simulink model "afe_inv_ttype_psm"  (R2026a)
settings: Solver=ode23tb  StopTime=simlength  FixedStep=tc  MaxStep=glb_time.tc
values from neighbouring files (symbols this model uses):
  afe_ctrl = ctrl_afe_setup(glb_time.ts_afe, grid_emu.omega_grid_nom)    [init_model.m]
  afe_pwm_phase_shift_mod1 = 0    [init_model.m]
  DThs_init = 0    [init_model.m]
  filters = setup_global_filters(glb_time.ts_afe, glb_time.ts_inv, glb_time.ts_dab, glb_time.tc)    [init_model.m]
  frt_data = frt_settings(test_index, test_subindex, asymmetric_error_type,      enable_frt_1, enable_frt_2, start_time_LVRT, deepPOSxi, deepPOSeta, deepNEGxi, deepNEGeta)    [init_model.m]
  glb_time = timing_setup(fpwm_afe, trgo_afe, fpwm_inv, trgo_inv, fpwm_single_phase_inv, trgo_single_phase_inv, fpwm_dab, trgo_dab,      fpwm_psfbc, trgo_psfbc, fpwm_isop_rail, trgo_isop_rail, fpwm_cllc, trgo_cllc, t_measure, tc_factor, tc_decimation, delay_pwm, dead_time_afe,      dead_time_inv, dead_time_single_phase_inv, dead_time_dab, dead_time_psfbc, dead_time_isop_rail, dead_time_cllc)    [init_model.m]
  grid_emu = grid_three_phase_emulator('Dyn11', delta_star, grid_nominal_power, application_voltage, us1, us2, fgrid,                  eq_grid_inductance, eq_grid_resistance, eta, ucc, i1m, p_iron, n1, n2, core_area, core_length, mur,                  up_xi_pu_ref, up_eta_pu_ref, un_xi_pu_ref, un_eta_pu_ref)    [init_model.m]
  i_react_pos_ref_2 = -ixi_ref_mod1*tan(acos(0.95))    [init_model.m]
  i_react_pos_ref_3 = ixi_ref_mod1*tan(acos(0.95))    [init_model.m]
  ixi_ref_mod1 = -0.85    [init_model.m]
  ki_align = 18    [init_model.m]
  kp_align = 0.25    [init_model.m]
  lim_down_align = -0.05    [init_model.m]
  lim_up_align = 0.05    [init_model.m]
  mavarage_filter_frequency_base_order = 2    [init_model.m]
  omega_m_sim = psm.omega_m_bez    [init_model.m]
  psm = psm_calculus()    [init_model.m]
  psm_ctrl = ctrl_pmsm_setup(glb_time.ts_inv, psm.omega_bez, u_psm_scale, psm.Jm_norm)    [init_model.m]
  simlength = 1.75    [init_model.m]
  Tambient = 40    [init_model.m]
  time_aux_power_supply_fault = 1e3    (= 1000)    [init_model.m]
  time_gain_afe_module_1 = 1.0002    [init_model.m]
  time_gain_inv_module_2 = 1.001    [init_model.m]
  time_i_react_pos_ref_1 = start_time_LVRT + error_length + 0.335    [init_model.m]
  time_i_react_pos_ref_2 = time_i_react_pos_ref_1 + 0.5    (= 0.5)    [init_model.m]
  time_start_motor_control = 0.25    [init_model.m]
  torque_overload_factor = 1    [init_model.m]
  u_cm_comp_mod1 = 0    [init_model.m]
  u_psm_scale_ekf = sqrt(3)/2 * 2/3 * hwdata.inv.udc_nom/psm.ubez    [init_model.m]
undefined symbols (not defined in the file or in its folder): hwdata, magnitude, omega_m_bez, rpm_base, torque_base
libraries: fl_lib x74, nesl_utility x43, moving_average_filter x10, moving_average_filter_cc x8, discrete_time_low_pass_filter x4, sl_discontinuities x3, single_phase_transformer_lib x3, linear_double_integrator_observer_ccaller x2, threephase_inductor_lib x2, dclink_for_three_levels x2, three_phase_three_level_ttype_inverter_ideal_switch_based_model x2, cstblocks_lti x2
(part 9 of 9)

== matlab function afe_inv_ttype_psm/afe_abc_inv_psm_mod1/inv_psm_mod1/inverter/deadtime_generator_for_ttype/dead_time_generator_cmos_simulink_phv/dead_time_leg_generator_1/MATLAB Function3 ==
  data: u input; y output; Vpos_rail_dtg parameter
function y = not_cmos(u, Vpos_rail_dtg)

vth = Vpos_rail_dtg/2;

if u > vth
    y = 0;
else
    y = Vpos_rail_dtg;
end

== matlab function afe_inv_ttype_psm/afe_abc_inv_psm_mod1/inv_psm_mod1/inverter/deadtime_generator_for_ttype/dead_time_generator_cmos_simulink_phv/dead_time_leg_generator_1/MATLAB Function4 ==
  data: u1 input; u2 input; y output; Vpos_rail_dtg parameter
function y = and_cmos(u1, u2, Vpos_rail_dtg)

vth = Vpos_rail_dtg/2;

if (u1 > vth && u2 > vth)
    y = Vpos_rail_dtg;
else
    y = 0;
end

== matlab function afe_inv_ttype_psm/afe_abc_inv_psm_mod1/inv_psm_mod1/inverter/deadtime_generator_for_ttype/dead_time_generator_cmos_simulink_phv/dead_time_leg_generator_1/MATLAB Function5 ==
  data: u1 input; u2 input; y output; Vpos_rail_dtg parameter
function y = and_cmos(u1, u2, Vpos_rail_dtg)

vth = Vpos_rail_dtg/2;

if (u1 > vth && u2 > vth)
    y = Vpos_rail_dtg;
else
    y = 0;
end

== matlab function afe_inv_ttype_psm/afe_abc_inv_psm_mod1/inv_psm_mod1/inverter/deadtime_generator_for_ttype/dead_time_generator_cmos_simulink_phv/dead_time_leg_generator_1/MATLAB Function6 ==
  data: u input; y output; Vpos_rail_dtg parameter
function y = not_cmos(u, Vpos_rail_dtg)

vth = Vpos_rail_dtg/2;

if u > vth
    y = 0;
else
    y = Vpos_rail_dtg;
end

== matlab function afe_inv_ttype_psm/afe_abc_inv_psm_mod1/inv_psm_mod1/inverter/deadtime_generator_for_ttype/dead_time_generator_cmos_simulink_phv/dead_time_leg_generator_1/MATLAB Function7 ==
  data: u input; y output; Vpos_rail_dtg parameter
function y = not_cmos(u, Vpos_rail_dtg)

vth = Vpos_rail_dtg/2;

if u > vth
    y = 0;
else
    y = Vpos_rail_dtg;
end

== matlab function afe_inv_ttype_psm/afe_abc_inv_psm_mod1/inv_psm_mod1/inverter/deadtime_generator_for_ttype/dead_time_generator_cmos_simulink_phv/dead_time_leg_generator_1/MATLAB Function8 ==
  data: u input; y output; Vpos_rail_dtg parameter
function y = not_cmos(u, Vpos_rail_dtg)

vth = Vpos_rail_dtg/2;

if u > vth
    y = 0;
else
    y = Vpos_rail_dtg;
end

== matlab function afe_inv_ttype_psm/afe_abc_inv_psm_mod1/inv_psm_mod1/inverter/deadtime_generator_for_ttype/dead_time_generator_cmos_simulink_phv/dead_time_leg_generator_1/MATLAB Function9 ==
  data: u1 input; u2 input; y output; Vpos_rail_dtg parameter
function y = and_cmos(u1, u2, Vpos_rail_dtg)

vth = Vpos_rail_dtg/2;

if (u1 > vth && u2 > vth)
    y = Vpos_rail_dtg;
else
    y = 0;
end

== matlab function afe_inv_ttype_psm/afe_abc_inv_psm_mod1/inv_psm_mod1/inverter/deadtime_generator_for_ttype/dead_time_generator_cmos_simulink_phw/dead_time_leg_generator_1/MATLAB Function ==
  data: u input; y output; Vpos_rail_dtg parameter
function y = not_cmos(u, Vpos_rail_dtg)

vth = Vpos_rail_dtg/2;

if u > vth
    y = 0;
else
    y = Vpos_rail_dtg;
end

== matlab function afe_inv_ttype_psm/afe_abc_inv_psm_mod1/inv_psm_mod1/inverter/deadtime_generator_for_ttype/dead_time_generator_cmos_simulink_phw/dead_time_leg_generator_1/MATLAB Function1 ==
  data: u1 input; u2 input; y output; Vpos_rail_dtg parameter
function y = and_cmos(u1, u2, Vpos_rail_dtg)

vth = Vpos_rail_dtg/2;

if (u1 > vth && u2 > vth)
    y = Vpos_rail_dtg;
else
    y = 0;
end

== matlab function afe_inv_ttype_psm/afe_abc_inv_psm_mod1/inv_psm_mod1/inverter/deadtime_generator_for_ttype/dead_time_generator_cmos_simulink_phw/dead_time_leg_generator_1/MATLAB Function2 ==
  data: u input; y output; Vpos_rail_dtg parameter
function y = not_cmos(u, Vpos_rail_dtg)

vth = Vpos_rail_dtg/2;

if u > vth
    y = 0;
else
    y = Vpos_rail_dtg;
end

== matlab function afe_inv_ttype_psm/afe_abc_inv_psm_mod1/inv_psm_mod1/inverter/deadtime_generator_for_ttype/dead_time_generator_cmos_simulink_phw/dead_time_leg_generator_1/MATLAB Function3 ==
  data: u input; y output; Vpos_rail_dtg parameter
function y = not_cmos(u, Vpos_rail_dtg)

vth = Vpos_rail_dtg/2;

if u > vth
    y = 0;
else
    y = Vpos_rail_dtg;
end

== matlab function afe_inv_ttype_psm/afe_abc_inv_psm_mod1/inv_psm_mod1/inverter/deadtime_generator_for_ttype/dead_time_generator_cmos_simulink_phw/dead_time_leg_generator_1/MATLAB Function4 ==
  data: u1 input; u2 input; y output; Vpos_rail_dtg parameter
function y = and_cmos(u1, u2, Vpos_rail_dtg)

vth = Vpos_rail_dtg/2;

if (u1 > vth && u2 > vth)
    y = Vpos_rail_dtg;
else
    y = 0;
end

== matlab function afe_inv_ttype_psm/afe_abc_inv_psm_mod1/inv_psm_mod1/inverter/deadtime_generator_for_ttype/dead_time_generator_cmos_simulink_phw/dead_time_leg_generator_1/MATLAB Function5 ==
  data: u1 input; u2 input; y output; Vpos_rail_dtg parameter
function y = and_cmos(u1, u2, Vpos_rail_dtg)

vth = Vpos_rail_dtg/2;

if (u1 > vth && u2 > vth)
    y = Vpos_rail_dtg;
else
    y = 0;
end

== matlab function afe_inv_ttype_psm/afe_abc_inv_psm_mod1/inv_psm_mod1/inverter/deadtime_generator_for_ttype/dead_time_generator_cmos_simulink_phu/dead_time_leg_generator_1/MATLAB Function ==
  data: u input; y output; Vpos_rail_dtg parameter
function y = not_cmos(u, Vpos_rail_dtg)

vth = Vpos_rail_dtg/2;

if u > vth
    y = 0;
else
    y = Vpos_rail_dtg;
end

== matlab function afe_inv_ttype_psm/afe_abc_inv_psm_mod1/inv_psm_mod1/inverter/deadtime_generator_for_ttype/dead_time_generator_cmos_simulink_phw/dead_time_leg_generator_1/MATLAB Function6 ==
  data: u input; y output; Vpos_rail_dtg parameter
function y = not_cmos(u, Vpos_rail_dtg)

vth = Vpos_rail_dtg/2;

if u > vth
    y = 0;
else
    y = Vpos_rail_dtg;
end

== matlab function afe_inv_ttype_psm/afe_abc_inv_psm_mod1/inv_psm_mod1/inverter/deadtime_generator_for_ttype/dead_time_generator_cmos_simulink_phw/dead_time_leg_generator_1/MATLAB Function7 ==
  data: u input; y output; Vpos_rail_dtg parameter
function y = not_cmos(u, Vpos_rail_dtg)

vth = Vpos_rail_dtg/2;

if u > vth
    y = 0;
else
    y = Vpos_rail_dtg;
end

== matlab function afe_inv_ttype_psm/afe_abc_inv_psm_mod1/inv_psm_mod1/inverter/deadtime_generator_for_ttype/dead_time_generator_cmos_simulink_phw/dead_time_leg_generator_1/MATLAB Function8 ==
  data: u input; y output; Vpos_rail_dtg parameter
function y = not_cmos(u, Vpos_rail_dtg)

vth = Vpos_rail_dtg/2;

if u > vth
    y = 0;
else
    y = Vpos_rail_dtg;
end

== matlab function afe_inv_ttype_psm/afe_abc_inv_psm_mod1/inv_psm_mod1/inverter/deadtime_generator_for_ttype/dead_time_generator_cmos_simulink_phw/dead_time_leg_generator_1/MATLAB Function9 ==
  data: u1 input; u2 input; y output; Vpos_rail_dtg parameter
function y = and_cmos(u1, u2, Vpos_rail_dtg)

vth = Vpos_rail_dtg/2;

if (u1 > vth && u2 > vth)
    y = Vpos_rail_dtg;
else
    y = 0;
end

== matlab function afe_inv_ttype_psm/afe_abc_inv_psm_mod1/inv_psm_mod1/inverter/timer/MATLAB Function ==
  data: t input; y output; phase input; period input
function y = ramp_up_down(t,phase,period)
x = sin(2*pi/period*t - phase -pi/2);
y = asin(x)/pi + 1/2;

== matlab function afe_inv_ttype_psm/afe_abc_inv_psm_mod1/inv_psm_mod1/inverter_ctrl/inverter_control/encoder-sensorless-switch/MATLAB Function ==
  data: omega_psm input; omega_ctrl output; phase_psm input; omega_obs input; phase_obs input; phase_ctrl output; omega_th input
function [omega_ctrl, phase_ctrl] = switch_enc2obs(omega_psm, phase_psm, omega_obs, phase_obs, omega_th)

if abs(omega_psm) > omega_th
    omega_ctrl = omega_obs;
    phase_ctrl = phase_obs;
else
    omega_ctrl = omega_psm;
    phase_ctrl = phase_psm;
end

== matlab function afe_inv_ttype_psm/afe_abc_inv_psm_mod1/inv_psm_mod1/inverter_ctrl/inverter_control/inner_ctrl/bemf_observer1/EKF_bemf_observer/extended_kalman_observer/double_integrator_observer/bounder1 ==
  data: u input; y output
function y = bounder(u)
    y = -pi + mod(u+3*pi,2*pi);
end

== matlab function afe_inv_ttype_psm/afe_abc_inv_psm_mod1/inv_psm_mod1/inverter_ctrl/inverter_control/inner_ctrl/bemf_observer1/EKF_bemf_observer/extended_kalman_observer/double_integrator_observer/bounder2 ==
  data: u input; y output
function y = bounder(u)
    y = -pi + mod(u+3*pi,2*pi);
end

== matlab function afe_inv_ttype_psm/afe_abc_inv_psm_mod1/inv_psm_mod1/inverter_ctrl/inverter_control/inner_ctrl/bemf_observer1/bemf_observer/double_integrator_observer/bounder1 ==
  data: u input; y output
function y = bounder(u)
    
    y = -pi + mod(u+3*pi,2*pi);
end

== matlab function afe_inv_ttype_psm/afe_abc_inv_psm_mod1/AFE_control/afe_control/current_ctrl/inner_current_ctrl/zero_current_ctrl/antiwind_up/MATLAB Function2 ==
  data: a input; alpha output; b input; c input; beta output; gamma output
function [alpha,beta, gamma] = abc2alphabeta(a,b,c)

alpha = 2/3*(a - 1/2*b - 1/2*c);
beta  = 1/sqrt(3)*(b - c);
gamma = (a+b+c)/3;

end

== matlab function afe_inv_ttype_psm/afe_abc_inv_psm_mod1/inv_psm_mod1/inverter_ctrl/inverter_control/inner_ctrl/bemf_observer1/bemf_observer/double_integrator_observer/bounder2 ==
  data: u input; y output
function y = bounder(u)
    
    u = -pi + mod(u+3*pi,2*pi);
    
    y = u;
end

== matlab function afe_inv_ttype_psm/afe_abc_inv_psm_mod1/inv_psm_mod1/inverter_ctrl/inverter_control/inner_ctrl/current_transformation/alphabeta2dq ==
  data: alpha input; d output; beta input; gamma input; q output
function [d,q] = alphabeta2dq(alpha,beta,gamma)

    d  =  alpha*cos(gamma) + beta*sin(gamma);
    q = -alpha*sin(gamma) + beta*cos(gamma);

end

== matlab function afe_inv_ttype_psm/afe_abc_inv_psm_mod1/inv_psm_mod1/inverter_ctrl/inverter_control/inner_ctrl/current_transformation/uvw2alphabeta ==
  data: u input; alpha output; v input; w input; beta output
function [alpha,beta] = uvw2alphabeta(u,v,w)

alpha = 2/3*(u - 1/2*v - 1/2*w);
beta  = 2/3*(sqrt(3)/2*(v - w));

end

== matlab function afe_inv_ttype_psm/afe_abc_inv_psm_mod1/afe/deadtime_generator_for_ttype/dead_time_generator_cmos_simulink_phu/dead_time_leg_generator_1/MATLAB Function ==
  data: u input; y output; Vpos_rail_dtg parameter
function y = not_cmos(u, Vpos_rail_dtg)

vth = Vpos_rail_dtg/2;

if u > vth
    y = 0;
else
    y = Vpos_rail_dtg;
end

== matlab function afe_inv_ttype_psm/afe_abc_inv_psm_mod1/afe/deadtime_generator_for_ttype/dead_time_generator_cmos_simulink_phu/dead_time_leg_generator_1/MATLAB Function1 ==
  data: u1 input; u2 input; y output; Vpos_rail_dtg parameter
function y = and_cmos(u1, u2, Vpos_rail_dtg)

vth = Vpos_rail_dtg/2;

if (u1 > vth && u2 > vth)
    y = Vpos_rail_dtg;
else
    y = 0;
end

== matlab function afe_inv_ttype_psm/afe_abc_inv_psm_mod1/afe/deadtime_generator_for_ttype/dead_time_generator_cmos_simulink_phu/dead_time_leg_generator_1/MATLAB Function2 ==
  data: u input; y output; Vpos_rail_dtg parameter
function y = not_cmos(u, Vpos_rail_dtg)

vth = Vpos_rail_dtg/2;

if u > vth
    y = 0;
else
    y = Vpos_rail_dtg;
end

== matlab function afe_inv_ttype_psm/afe_abc_inv_psm_mod1/afe/deadtime_generator_for_ttype/dead_time_generator_cmos_simulink_phu/dead_time_leg_generator_1/MATLAB Function3 ==
  data: u input; y output; Vpos_rail_dtg parameter
function y = not_cmos(u, Vpos_rail_dtg)

vth = Vpos_rail_dtg/2;

if u > vth
    y = 0;
else
    y = Vpos_rail_dtg;
end

== matlab function afe_inv_ttype_psm/afe_abc_inv_psm_mod1/afe/deadtime_generator_for_ttype/dead_time_generator_cmos_simulink_phu/dead_time_leg_generator_1/MATLAB Function4 ==
  data: u1 input; u2 input; y output; Vpos_rail_dtg parameter
function y = and_cmos(u1, u2, Vpos_rail_dtg)

vth = Vpos_rail_dtg/2;

if (u1 > vth && u2 > vth)
    y = Vpos_rail_dtg;
else
    y = 0;
end

== matlab function afe_inv_ttype_psm/afe_abc_inv_psm_mod1/afe/deadtime_generator_for_ttype/dead_time_generator_cmos_simulink_phu/dead_time_leg_generator_1/MATLAB Function5 ==
  data: u1 input; u2 input; y output; Vpos_rail_dtg parameter
function y = and_cmos(u1, u2, Vpos_rail_dtg)

vth = Vpos_rail_dtg/2;

if (u1 > vth && u2 > vth)
    y = Vpos_rail_dtg;
else
    y = 0;
end

== matlab function afe_inv_ttype_psm/afe_abc_inv_psm_mod1/afe/deadtime_generator_for_ttype/dead_time_generator_cmos_simulink_phu/dead_time_leg_generator_1/MATLAB Function6 ==
  data: u input; y output; Vpos_rail_dtg parameter
function y = not_cmos(u, Vpos_rail_dtg)

vth = Vpos_rail_dtg/2;

if u > vth
    y = 0;
else
    y = Vpos_rail_dtg;
end

== matlab function afe_inv_ttype_psm/afe_abc_inv_psm_mod1/afe/deadtime_generator_for_ttype/dead_time_generator_cmos_simulink_phu/dead_time_leg_generator_1/MATLAB Function7 ==
  data: u input; y output; Vpos_rail_dtg parameter
function y = not_cmos(u, Vpos_rail_dtg)

vth = Vpos_rail_dtg/2;

if u > vth
    y = 0;
else
    y = Vpos_rail_dtg;
end

== matlab function afe_inv_ttype_psm/afe_abc_inv_psm_mod1/afe/deadtime_generator_for_ttype/dead_time_generator_cmos_simulink_phu/dead_time_leg_generator_1/MATLAB Function8 ==
  data: u input; y output; Vpos_rail_dtg parameter
function y = not_cmos(u, Vpos_rail_dtg)

vth = Vpos_rail_dtg/2;

if u > vth
    y = 0;
else
    y = Vpos_rail_dtg;
end

== matlab function afe_inv_ttype_psm/afe_abc_inv_psm_mod1/afe/deadtime_generator_for_ttype/dead_time_generator_cmos_simulink_phu/dead_time_leg_generator_1/MATLAB Function9 ==
  data: u1 input; u2 input; y output; Vpos_rail_dtg parameter
function y = and_cmos(u1, u2, Vpos_rail_dtg)

vth = Vpos_rail_dtg/2;

if (u1 > vth && u2 > vth)
    y = Vpos_rail_dtg;
else
    y = 0;
end

== matlab function afe_inv_ttype_psm/afe_abc_inv_psm_mod1/AFE_control/afe_control/grid_voltage_phase_lock_loops/FHT-PLL/pll_stageA/filter_and_transformation/abc2alphabeta ==
  data: a input; alpha output; b input; c input; beta output
function [alpha,beta] = abc2alphabeta(a,b,c)

alpha = 2/3*(a - 1/2*b - 1/2*c);
beta  = 1/sqrt(3)*(b - c);

end

== matlab function afe_inv_ttype_psm/afe_abc_inv_psm_mod1/afe/deadtime_generator_for_ttype/dead_time_generator_cmos_simulink_phv/dead_time_leg_generator_1/MATLAB Function ==
  data: u input; y output; Vpos_rail_dtg parameter
function y = not_cmos(u, Vpos_rail_dtg)

vth = Vpos_rail_dtg/2;

if u > vth
    y = 0;
else
    y = Vpos_rail_dtg;
end

== matlab function afe_inv_ttype_psm/afe_abc_inv_psm_mod1/afe/deadtime_generator_for_ttype/dead_time_generator_cmos_simulink_phv/dead_time_leg_generator_1/MATLAB Function1 ==
  data: u1 input; u2 input; y output; Vpos_rail_dtg parameter
function y = and_cmos(u1, u2, Vpos_rail_dtg)

vth = Vpos_rail_dtg/2;

if (u1 > vth && u2 > vth)
    y = Vpos_rail_dtg;
else
    y = 0;
end

== matlab function afe_inv_ttype_psm/afe_abc_inv_psm_mod1/afe/deadtime_generator_for_ttype/dead_time_generator_cmos_simulink_phv/dead_time_leg_generator_1/MATLAB Function2 ==
  data: u input; y output; Vpos_rail_dtg parameter
function y = not_cmos(u, Vpos_rail_dtg)

vth = Vpos_rail_dtg/2;

if u > vth
    y = 0;
else
    y = Vpos_rail_dtg;
end

== matlab function afe_inv_ttype_psm/afe_abc_inv_psm_mod1/afe/deadtime_generator_for_ttype/dead_time_generator_cmos_simulink_phv/dead_time_leg_generator_1/MATLAB Function3 ==
  data: u input; y output; Vpos_rail_dtg parameter
function y = not_cmos(u, Vpos_rail_dtg)

vth = Vpos_rail_dtg/2;

if u > vth
    y = 0;
else
    y = Vpos_rail_dtg;
end

== matlab function afe_inv_ttype_psm/afe_abc_inv_psm_mod1/afe/deadtime_generator_for_ttype/dead_time_generator_cmos_simulink_phv/dead_time_leg_generator_1/MATLAB Function4 ==
  data: u1 input; u2 input; y output; Vpos_rail_dtg parameter
function y = and_cmos(u1, u2, Vpos_rail_dtg)

vth = Vpos_rail_dtg/2;

if (u1 > vth && u2 > vth)
    y = Vpos_rail_dtg;
else
    y = 0;
end

== matlab function afe_inv_ttype_psm/afe_abc_inv_psm_mod1/afe/deadtime_generator_for_ttype/dead_time_generator_cmos_simulink_phv/dead_time_leg_generator_1/MATLAB Function5 ==
  data: u1 input; u2 input; y output; Vpos_rail_dtg parameter
function y = and_cmos(u1, u2, Vpos_rail_dtg)

vth = Vpos_rail_dtg/2;

if (u1 > vth && u2 > vth)
    y = Vpos_rail_dtg;
else
    y = 0;
end

== matlab function afe_inv_ttype_psm/afe_abc_inv_psm_mod1/afe/deadtime_generator_for_ttype/dead_time_generator_cmos_simulink_phv/dead_time_leg_generator_1/MATLAB Function6 ==
  data: u input; y output; Vpos_rail_dtg parameter
function y = not_cmos(u, Vpos_rail_dtg)

vth = Vpos_rail_dtg/2;

if u > vth
    y = 0;
else
    y = Vpos_rail_dtg;
end

== matlab function afe_inv_ttype_psm/afe_abc_inv_psm_mod1/afe/deadtime_generator_for_ttype/dead_time_generator_cmos_simulink_phv/dead_time_leg_generator_1/MATLAB Function7 ==
  data: u input; y output; Vpos_rail_dtg parameter
function y = not_cmos(u, Vpos_rail_dtg)

vth = Vpos_rail_dtg/2;

if u > vth
    y = 0;
else
    y = Vpos_rail_dtg;
end

== matlab function afe_inv_ttype_psm/afe_abc_inv_psm_mod1/afe/deadtime_generator_for_ttype/dead_time_generator_cmos_simulink_phv/dead_time_leg_generator_1/MATLAB Function8 ==
  data: u input; y output; Vpos_rail_dtg parameter
function y = not_cmos(u, Vpos_rail_dtg)

vth = Vpos_rail_dtg/2;

if u > vth
    y = 0;
else
    y = Vpos_rail_dtg;
end

== matlab function afe_inv_ttype_psm/afe_abc_inv_psm_mod1/afe/deadtime_generator_for_ttype/dead_time_generator_cmos_simulink_phv/dead_time_leg_generator_1/MATLAB Function9 ==
  data: u1 input; u2 input; y output; Vpos_rail_dtg parameter
function y = and_cmos(u1, u2, Vpos_rail_dtg)

vth = Vpos_rail_dtg/2;

if (u1 > vth && u2 > vth)
    y = Vpos_rail_dtg;
else
    y = 0;
end

== matlab function afe_inv_ttype_psm/afe_abc_inv_psm_mod1/afe/deadtime_generator_for_ttype/dead_time_generator_cmos_simulink_phw/dead_time_leg_generator_1/MATLAB Function ==
  data: u input; y output; Vpos_rail_dtg parameter
function y = not_cmos(u, Vpos_rail_dtg)

vth = Vpos_rail_dtg/2;

if u > vth
    y = 0;
else
    y = Vpos_rail_dtg;
end

== matlab function afe_inv_ttype_psm/afe_abc_inv_psm_mod1/afe/deadtime_generator_for_ttype/dead_time_generator_cmos_simulink_phw/dead_time_leg_generator_1/MATLAB Function1 ==
  data: u1 input; u2 input; y output; Vpos_rail_dtg parameter
function y = and_cmos(u1, u2, Vpos_rail_dtg)

vth = Vpos_rail_dtg/2;

if (u1 > vth && u2 > vth)
    y = Vpos_rail_dtg;
else
    y = 0;
end

== matlab function afe_inv_ttype_psm/afe_abc_inv_psm_mod1/AFE_control/afe_control/grid_voltage_phase_lock_loops/FHT-PLL/pll_stageA/sequences/alphabeta2xieta ==
  data: alpha input; xi output; beta input; gamma input; eta output
function [xi,eta] = alphabeta2xieta_pos(alpha,beta,gamma)

    xi  =  (alpha*cos(gamma) + beta*sin(gamma));
    eta = (-alpha*sin(gamma) + beta*cos(gamma));

end

== matlab function afe_inv_ttype_psm/afe_abc_inv_psm_mod1/afe/deadtime_generator_for_ttype/dead_time_generator_cmos_simulink_phw/dead_time_leg_generator_1/MATLAB Function2 ==
  data: u input; y output; Vpos_rail_dtg parameter
function y = not_cmos(u, Vpos_rail_dtg)

vth = Vpos_rail_dtg/2;

if u > vth
    y = 0;
else
    y = Vpos_rail_dtg;
end

== matlab function afe_inv_ttype_psm/afe_abc_inv_psm_mod1/afe/deadtime_generator_for_ttype/dead_time_generator_cmos_simulink_phw/dead_time_leg_generator_1/MATLAB Function3 ==
  data: u input; y output; Vpos_rail_dtg parameter
function y = not_cmos(u, Vpos_rail_dtg)

vth = Vpos_rail_dtg/2;

if u > vth
    y = 0;
else
    y = Vpos_rail_dtg;
end

== matlab function afe_inv_ttype_psm/afe_abc_inv_psm_mod1/afe/deadtime_generator_for_ttype/dead_time_generator_cmos_simulink_phw/dead_time_leg_generator_1/MATLAB Function4 ==
  data: u1 input; u2 input; y output; Vpos_rail_dtg parameter
function y = and_cmos(u1, u2, Vpos_rail_dtg)

vth = Vpos_rail_dtg/2;

if (u1 > vth && u2 > vth)
    y = Vpos_rail_dtg;
else
    y = 0;
end

== matlab function afe_inv_ttype_psm/afe_abc_inv_psm_mod1/afe/deadtime_generator_for_ttype/dead_time_generator_cmos_simulink_phw/dead_time_leg_generator_1/MATLAB Function5 ==
  data: u1 input; u2 input; y output; Vpos_rail_dtg parameter
function y = and_cmos(u1, u2, Vpos_rail_dtg)

vth = Vpos_rail_dtg/2;

if (u1 > vth && u2 > vth)
    y = Vpos_rail_dtg;
else
    y = 0;
end

== matlab function afe_inv_ttype_psm/afe_abc_inv_psm_mod1/afe/deadtime_generator_for_ttype/dead_time_generator_cmos_simulink_phw/dead_time_leg_generator_1/MATLAB Function6 ==
  data: u input; y output; Vpos_rail_dtg parameter
function y = not_cmos(u, Vpos_rail_dtg)

vth = Vpos_rail_dtg/2;

if u > vth
    y = 0;
else
    y = Vpos_rail_dtg;
end

== matlab function afe_inv_ttype_psm/afe_abc_inv_psm_mod1/afe/deadtime_generator_for_ttype/dead_time_generator_cmos_simulink_phw/dead_time_leg_generator_1/MATLAB Function7 ==
  data: u input; y output; Vpos_rail_dtg parameter
function y = not_cmos(u, Vpos_rail_dtg)

vth = Vpos_rail_dtg/2;

if u > vth
    y = 0;
else
    y = Vpos_rail_dtg;
end

== matlab function afe_inv_ttype_psm/afe_abc_inv_psm_mod1/afe/deadtime_generator_for_ttype/dead_time_generator_cmos_simulink_phw/dead_time_leg_generator_1/MATLAB Function8 ==
  data: u input; y output; Vpos_rail_dtg parameter
function y = not_cmos(u, Vpos_rail_dtg)

vth = Vpos_rail_dtg/2;

if u > vth
    y = 0;
else
    y = Vpos_rail_dtg;
end

== matlab function afe_inv_ttype_psm/afe_abc_inv_psm_mod1/afe/deadtime_generator_for_ttype/dead_time_generator_cmos_simulink_phw/dead_time_leg_generator_1/MATLAB Function9 ==
  data: u1 input; u2 input; y output; Vpos_rail_dtg parameter
function y = and_cmos(u1, u2, Vpos_rail_dtg)

vth = Vpos_rail_dtg/2;

if (u1 > vth && u2 > vth)
    y = Vpos_rail_dtg;
else
    y = 0;
end

== matlab function afe_inv_ttype_psm/afe_abc_inv_psm_mod1/inv_psm_mod1/inverter_ctrl/inverter_control/inner_ctrl/mp control/mpc_pu_d ==
  data: S1a output; S2a output; S3a output; S4a output; S1b output; S2b output; S3b output; S4b output; S1c output; S2c output; S3c output; S4c output; vdc1 input; vdc2 input; ialpha_ref input; ibeta_ref input; ialpha input; ualpha output; ibeta input; omega_hat input; psi_alpha_hat input; psi_beta_hat input; ubeta output; Lalpha_norm input; Rs_norm input; Lbeta_norm input; omega_bez input; k_kalman input; k_dc input; k_sw input; ts_inv input
function [S1a, S2a, S3a, S4a, S1b, S2b, S3b, S4b, S1c, S2c, S3c, S4c, ualpha, ubeta] = mpc_ttype_gate(...
    vdc1, vdc2, ialpha_ref, ibeta_ref, ialpha, ibeta, ...
    omega_hat, psi_alpha_hat, psi_beta_hat, Lalpha_norm, Rs_norm, Lbeta_norm, ...
omega_bez, k_kalman, k_dc, k_sw, ts_inv)
    
    % vdc1, vdc2: tensioni dei due condensatori (superiore e inferiore)
    % k_dc: peso per il bilanciamento del punto neutro nella funzione di costo
    
    persistent ualpha_prev ubeta_prev states_table
    
    if isempty(ualpha_prev)
        ualpha_prev = 0.0;
        ubeta_prev = 0.0;
        % Tabella dei 27 stati di commutazione [-1, 0, 1]
        states_table = [
            -1,-1,-1; -1,-1, 0; -1,-1, 1; -1, 0,-1; -1, 0, 0; -1, 0, 1; -1, 1,-1; -1, 1, 0; -1, 1, 1;
             0,-1,-1;  0,-1, 0;  0,-1, 1;  0, 0,-1;  0, 0, 0;  0, 0, 1;  0, 1,-1;  0, 1, 0;  0, 1, 1;
             1,-1,-1;  1,-1, 0;  1,-1, 1;  1, 0,-1;  1, 0, 0;  1, 0, 1;  1, 1,-1;  1, 1, 0;  1, 1, 1
        ];
    end

    Vdd = 15;
    ts = ts_inv * omega_bez;
    vdc_tot = vdc1 + vdc2;
    Vdc3 = vdc_tot / 3.0; 
    sqrt3_2 = 0.866025403784439;
    
    % Trasformazione inversa di Clarke per ottenere le correnti di fase attuali
    % Necessarie per calcolare la corrente del punto neutro i_np
    ia = ialpha;
    ib = -0.5 * ialpha + sqrt3_2 * ibeta;
    ic = -0.5 * ialpha - sqrt3_2 * ibeta;

    minJ = 1e18; 
    best_idx = 14; 
    ualpha = 0.0;
    ubeta = 0.0;

    for n = 1:27
        % 1. Tensioni candidate
        sa = states_table(n,1);
        sb = states_table(n,2);
        sc = states_table(n,3);
        
        ua = Vdc3 * (sa - 0.5*sb - 0.5*sc);
        ub = Vdc3 * (sqrt3_2 * sb - sqrt3_2 * sc);

        % 2. Predizione correnti
        ia_p = (1.0 - Rs_norm/Lalpha_norm*ts)*ialpha + (omega_hat/Lalpha_norm*psi_beta_hat*ts) + (ua*ts/Lalpha_norm);
        ib_p = (1.0 - Rs_norm/Lbeta_norm*ts)*ibeta - (omega_hat/Lbeta_norm*psi_alpha_hat*ts) + (ub*ts/Lbeta_norm);

        % 3. Bilanciamento Punto Neutro
        % La corrente che esce dal punto neutro (np) è data dalle fasi che sono nello stato '0'
        % i_np = (sa==0)*ia + (sb==0)*ib + (sc==0)*ic
        inp = double(sa==0)*ia + double(sb==0)*ib + double(sc==0)*ic;
        
        % Predizione dello sbilanciamento futuro (delta_v = vdc1 - vdc2)
        % Se inp > 0, il punto neutro si scarica, influenzando la differenza tra i condensatori
        % Assumendo C1 = C2 = C, la variazione della differenza di tensione è proporzionale a inp
        dv_future = (vdc1 - vdc2) + (1/1e-3) * inp * ts; % 1e-3 è una capacità fittizia, k_dc compenserà

        % 4. Funzione di Costo
        J_error = k_kalman * ((ialpha_ref - ia_p)^2 + (ibeta_ref - ib_p)^2);
        J_sw = k_sw * ((ua - ualpha_prev)^2 + (ub - ubeta_prev)^2);
        J_dc = k_dc * (dv_future^2); % Termine di bilanciamento
        
        current_J = J_error + J_sw + J_dc;

        if current_J < minJ
            minJ = current_J;
            best_idx = n;
            ualpha = ua;
            ubeta = ub;
        end
    end

    ualpha_prev = ualpha;
    ubeta_prev = ubeta;

    % Decodifica Gate (identica a prima)
    ga = states_table(best_idx, 1);
    gb = states_table(best_idx, 2);
    gc = states_table(best_idx, 3);

    S1a = Vdd * double(ga == 1); S2a = Vdd * double(ga >= 0); S3a = Vdd * double(ga <= 0); S4a = Vdd * double(ga == -1);
    S1b = Vdd * double(gb == 1); S2b = Vdd * double(gb >= 0); S3b = Vdd * double(gb <= 0); S4b = Vdd * double(gb == -1);
    S1c = Vdd * double(gc == 1); S2c = Vdd * double(gc >= 0); S3c = Vdd * double(gc <= 0); S4c = Vdd * double(gc == -1);
end
